simulink model "test"  (R2022a)
settings: Solver=ode3  StartTime=0.0  StopTime=inf  RelTol=1e-3  EnableMultiTasking=on
libraries: arduinolib x1
settings Model: FPTRunName=Active  ExtModeTrigDuration=2  Creator=budea  LastModifiedBy=ix_andrei
settings SolverCC: AlgebraicLoopSolver=TrustRegion
settings DataIOCC: LimitDataPoints=on  SaveFormat=Array
settings OptimizationCC: ExpressionDepthLimit=2147483647  LifeSpan=Inf  MaxStackSize=64
settings DebuggingCC: UnderspecifiedInitializationDetection=Classic  MergeDetectMultiDrivingBlocksExec=none  FcnCallInpInsideContextMsg=warning  UnconnectedInputMsg=warning  UnconnectedOutputMsg=warning  UnconnectedLineMsg=warning  AllowSymbolicDim=off  StateNameClashWarn=warning  SFUnexpectedBacktrackingDiag=warning  SFNoUnconditionalDefaultTransitionDiag=warning  SFExecutionAtInitializationDiag=none  SFMachineParentedDataDiag=warning  ArithmeticOperatorsInVariantConditions=warning
settings HardwareCC: ProdBitPerPointer=32  ProdBitPerSizeT=32  ProdBitPerPtrDiffT=32  ProdLargestAtomicInteger=Long  ProdLargestAtomicFloat=Double  ProdWordSize=32  ProdHWDeviceType=ARM Compatible->ARM Cortex  UseEmbeddedCoderFeatures=off  UseSimulinkCoderFeatures=off
settings ModelReferenceCC: PropagateSignalLabelsOutOfModel=off
settings SFSimCC: SimUseLocalCustomCode=off  CustomCodeUndefinedFunction=UseInterfaceOnly
settings RTWCC: SystemTargetFile=ert.tlc  HardwareBoard=Arduino MKR1000  TemplateMakefile=ert_default_tmf  GenerateReport=on  RTWVerbose=off  RTWUseLocalCustomCode=off  Toolchain=Arduino ARM  BuildConfiguration=Faster Runs  LaunchReport=on  DLArmComputeVersion=19.05
settings CodeAppCC: ForceParamTrailComments=on  OperatorAnnotations=on  MangleLength=10  StateflowObjectComments=on  MATLABSourceComments=on
settings ERTTargetCC: MultiwordLength=2048  ERTCustomFileBanners=off  SupportContinuousTime=on  SupportNonInlinedSFcns=on  RemoveResetFunc=off  SupportVariableSizeSignals=on  ModelStepFunctionPrototypeControlCompliant=off  ExtModeTransport=3  ExtModeStaticAlloc=on  ExtModeStaticAllocSize=8192  ExtModeMexFile=ext_xcp  ExtModeIntrfLevel=Level2 - Open
settings ConfigComp: CovMetricSettings=dw  CovSaveCumulativeToWorkspaceVar=on  CovSaveSingleToWorkspaceVar=on  CovExternalEMLEnable=off  CovSFcnEnable=off

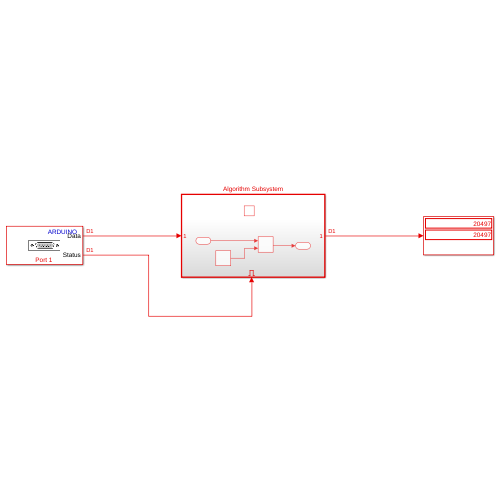
[thumbnail: Simulink's stored preview of the top-level diagram]
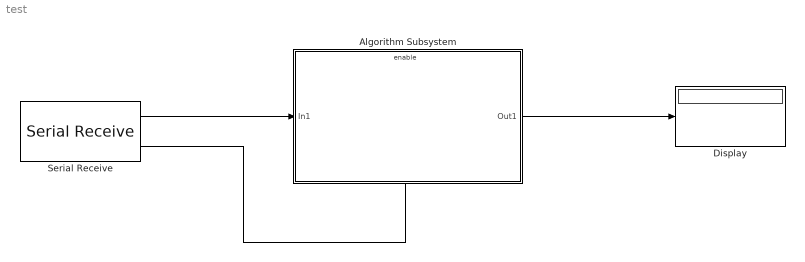
== system test ==
  Algorithm Subsystem : Subsystem
  Display : Display
      settings: Format=hex (Stored Integer)
  Serial Receive : arduinolib/Serial Receive  isARMArch=on  portNumber=1  DataType=uint8  Datalength=2  SampleTime=0.1  showOutStatus=on  blockPlatform=arduino
      settings: SourceProductBaseCode=ARDUINO
  wires:
  Serial Receive/2 -> Algorithm Subsystem/Enable
  Serial Receive/1 -> Algorithm Subsystem/1(In1)
  Algorithm Subsystem/1(Out1) -> Display/1

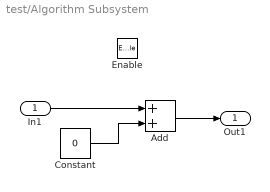
== system test/Algorithm Subsystem ==
  In1 : Inport
  Enable : EnablePort
  Add : Sum
  Constant : Constant  Value=0  SampleTime=-1
  Out1 : Outport  VectorParamsAs1DForOutWhenUnconnected=off
  wires:
  In1/1 -> Add/1
  Add/1 -> Out1/1
  Constant/1 -> Add/2
